simulink model "rns_sm"  (R2025b)
settings: Solver=ode45  StartTime=0.0  StopTime=T_END  MaxStep=0.01  RelTol=1e-10  AbsTol=1e-12
values from neighbouring files (symbols this model uses):
  a0 = 1    [run_rns_simscape.m]
  b0 = [a0/2 0]    [run_rns_simscape.m]
  I0 = m0*(a0^2 + a0^2)/12    (= 16.6666666667)    [run_rns_simscape.m]
  IN = MS.*LEN.^2/12    [run_rns_simscape.m]
  K_TH = 1.0    (= 1)    [run_rns_simscape.m]
  KP_EE = 2.0    (= 2)    [run_rns_simscape.m]
  LAM = 0.02    [run_rns_simscape.m]
  LEN = [1 1 0.5]    [run_rns_simscape.m]
  m = modelName    [build_rns_sm.m]
  m0 = 100    [run_rns_simscape.m]
  METHOD = cases{c, 2}    [run_rns_simscape.m]
  MS = [10 10 5]    [run_rns_simscape.m]
  QM0 = deg2rad([30 60 -45])    [run_rns_simscape.m]
  s = 10*x^3 - 15*x^4 + 6*x^5    [rns_controller.m]
  T_MOVE = 8    [run_rns_simscape.m]
  XG = goals.(cases{c, 1})    [run_rns_simscape.m]
  XS = d0(2:3).'    [run_rns_simscape.m]
  Y = squeeze(out.Y_sm)    [run_rns_simscape.m]
undefined symbols (not defined in the file or in its folder): X, Z
libraries: sm_lib x16, nesl_utility x10
settings Model: Creator=avaza  LastModifiedBy=avaza
settings DataIOCC: SaveOutput=off  TimeSaveName=t_sm  OutputOption=SpecifiedOutputTimes  OutputTimes=0:0.01:T_END
settings DebuggingCC: AlgebraicLoopMsg=none

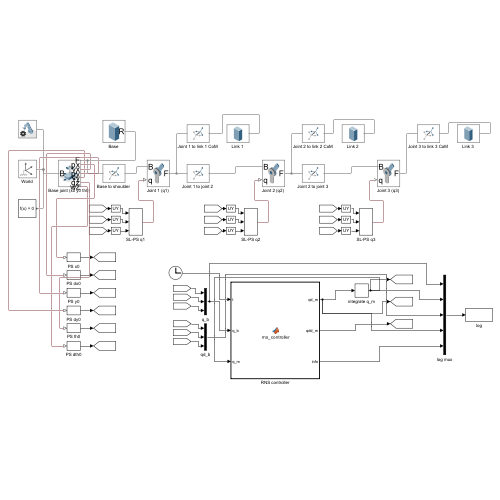
[thumbnail: Simulink's stored preview of the top-level diagram]
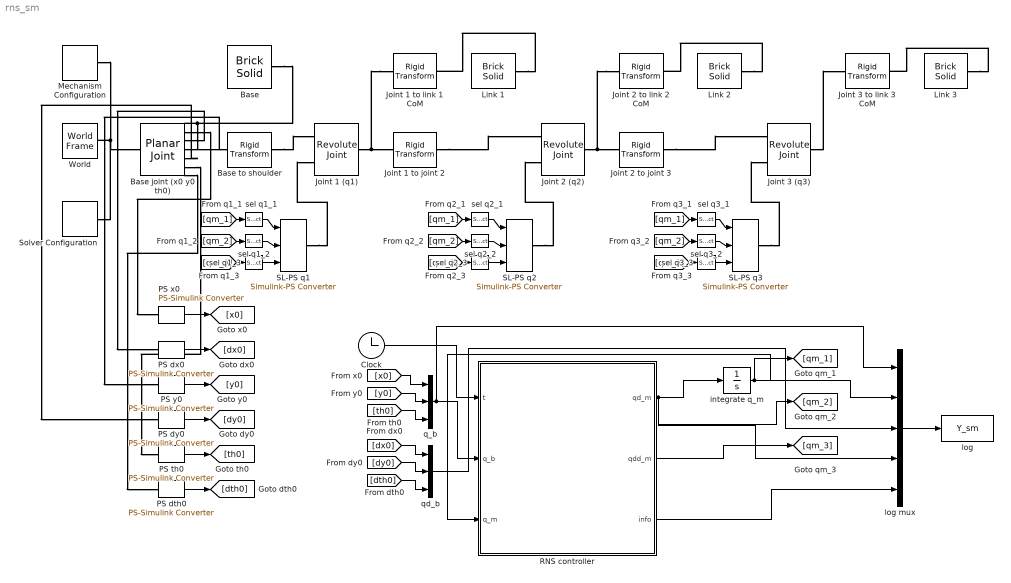
== system rns_sm ==
  Base : sm_lib/Body Elements/Brick Solid  BrickDimensions=[a0 a0 0.2]  BrickDimensionsUnits=m  ExportEntireGeometry=off  InertiaType=Custom  BasedOnType=Density  Density=1000  DensityUnits=kg/m^3  Mass=m0  MassUnits=kg  CenterOfMass=[0 0 0]  CenterOfMassUnits=m  MomentsOfInertia=[0.55*I0 0.55*I0 I0]  MomentsOfInertiaUnits=kg*m^2  ProductsOfInertia=[0 0 0]  ProductsOfInertiaUnits=kg*m^2  GraphicType=FromGeometry  MarkerShape=Sphere  MarkerSize=10  GraphicVisPropType=SimpleVisualProperties  GraphicDiffuseColor=[0.6 0.6 0.7]  GraphicOpacity=1  GraphicSpecularColor=[0.5 0.5 0.5 1.0]  GraphicAmbientColor=[0.15 0.15 0.15 1.0]  GraphicEmissiveColor=[0.0 0.0 0.0 1.0]  GraphicShininess=75  DoExposeReferenceFrame=on  SerializedFrames=<Frames/>
  Base joint (x0 y0 th0) : sm_lib/Joints/Planar Joint  JointMode=Normal  CompositeWrenchDir=FollowerOnBase  CompositeWrenchFrame=BaseFrame  SenseConstraintForce=off  SenseConstraintTorque=off  SenseTotalForce=off  SenseTotalTorque=off  PxPositionTargetSpecify=off  PxPositionTargetPriority=High  PxPositionTargetValue=0  PxPositionTargetValueUnits=m  PxVelocityTargetSpecify=off  PxVelocityTargetPriority=High  PxVelocityTargetValue=0  PxVelocityTargetValueUnits=m/s  PxEquilibriumPosition=0  PxEquilibriumPositionUnits=m  PxSpringStiffness=0  PxSpringStiffnessUnits=N/m  PxDampingCoefficient=0  PxDampingCoefficientUnits=N/(m/s)  PxLowerLimitSpecify=off  PxLowerLimitBound=-1  PxLowerLimitBoundUnits=m  PxLowerLimitStiffness=1e6  PxLowerLimitStiffnessUnits=N/m  PxLowerLimitDamping=1e3  PxLowerLimitDampingUnits=N/(m/s)  PxLowerLimitTransitionRegionWidth=1e-4  PxLowerLimitTransitionRegionWidthUnits=m  PxUpperLimitSpecify=off  PxUpperLimitBound=1  PxUpperLimitBoundUnits=m  PxUpperLimitStiffness=1e6  PxUpperLimitStiffnessUnits=N/m  PxUpperLimitDamping=1e3  PxUpperLimitDampingUnits=N/(m/s)  PxUpperLimitTransitionRegionWidth=1e-4  PxUpperLimitTransitionRegionWidthUnits=m  PxTorqueActuationMode=NoTorque  PxMotionActuationMode=ComputedMotion  PxSensePosition=on  PxSenseVelocity=on  PxSenseAcceleration=off  PxSenseTorqueForce=off  PxSenseLowerLimitTorqueForce=off  PxSenseUpperLimitTorqueForce=off  PyPositionTargetSpecify=off  PyPositionTargetPriority=High  PyPositionTargetValue=0  PyPositionTargetValueUnits=m  PyVelocityTargetSpecify=off  PyVelocityTargetPriority=High  PyVelocityTargetValue=0  PyVelocityTargetValueUnits=m/s  PyEquilibriumPosition=0  PyEquilibriumPositionUnits=m  PySpringStiffness=0  PySpringStiffnessUnits=N/m  PyDampingCoefficient=0  PyDampingCoefficientUnits=N/(m/s)  PyLowerLimitSpecify=off  PyLowerLimitBound=-1  PyLowerLimitBoundUnits=m  PyLowerLimitStiffness=1e6  PyLowerLimitStiffnessUnits=N/m  PyLowerLimitDamping=1e3  PyLowerLimitDampingUnits=N/(m/s)  PyLowerLimitTransitionRegionWidth=1e-4  PyLowerLimitTransitionRegionWidthUnits=m  PyUpperLimitSpecify=off  PyUpperLimitBound=1  PyUpperLimitBoundUnits=m  PyUpperLimitStiffness=1e6  PyUpperLimitStiffnessUnits=N/m  PyUpperLimitDamping=1e3  PyUpperLimitDampingUnits=N/(m/s)  PyUpperLimitTransitionRegionWidth=1e-4  PyUpperLimitTransitionRegionWidthUnits=m  PyTorqueActuationMode=NoTorque  PyMotionActuationMode=ComputedMotion  PySensePosition=on  PySenseVelocity=on  PySenseAcceleration=off  PySenseTorqueForce=off  PySenseLowerLimitTorqueForce=off  PySenseUpperLimitTorqueForce=off  RzPositionTargetSpecify=off  RzPositionTargetPriority=High  RzPositionTargetValue=0  RzPositionTargetValueUnits=deg  RzVelocityTargetSpecify=off  RzVelocityTargetPriority=High  RzVelocityTargetValue=0  RzVelocityTargetValueUnits=deg/s  RzEquilibriumPosition=0  RzEquilibriumPositionUnits=deg  RzSpringStiffness=0  RzSpringStiffnessUnits=N*m/deg  RzDampingCoefficient=0  RzDampingCoefficientUnits=N*m/(deg/s)  RzLowerLimitSpecify=off  RzLowerLimitBound=-90  RzLowerLimitBoundUnits=deg  RzLowerLimitStiffness=1e4  RzLowerLimitStiffnessUnits=N*m/deg  RzLowerLimitDamping=10  RzLowerLimitDampingUnits=N*m/(deg/s)  RzLowerLimitTransitionRegionWidth=0.1  RzLowerLimitTransitionRegionWidthUnits=deg  RzUpperLimitSpecify=off  RzUpperLimitBound=90  RzUpperLimitBoundUnits=deg  RzUpperLimitStiffness=1e4  RzUpperLimitStiffnessUnits=N*m/deg  RzUpperLimitDamping=10  RzUpperLimitDampingUnits=N*m/(deg/s)  RzUpperLimitTransitionRegionWidth=0.1  RzUpperLimitTransitionRegionWidthUnits=deg  RzTorqueActuationMode=NoTorque  RzMotionActuationMode=ComputedMotion  RzSensePosition=on  RzSenseVelocity=on  RzSenseAcceleration=off  RzSenseTorqueForce=off  RzSenseLowerLimitTorqueForce=off  RzSenseUpperLimitTorqueForce=off
  Base to shoulder : sm_lib/Frames and Transforms/Rigid Transform  RotationMethod=None  FollAlignAxisA=+X  BaseAlignAxisA=+Y  FollAlignAxisB=+Y  BaseAlignAxisB=+Z  RotationStandardAxis=+Z  RotationAngle=0  RotationAngleUnits=deg  RotationArbitraryAxis=[0 0 1]  RotationSequenceAxes=FollowerAxes  RotationSequence=XYX  RotationSequenceAngles=[0 0 0]  RotationSequenceAnglesUnits=deg  RotationMatrix=[1 0 0;0 1 0;0 0 1]  Quaternion=[1 0 0 0]  TranslationMethod=Cartesian  TranslationCartesianOffset=[b0(1) b0(2) 0]  TranslationCartesianOffsetUnits=m  TranslationStandardAxis=+Z  TranslationStandardOffset=0  TranslationStandardOffsetUnits=m  TranslationROffset=0  TranslationROffsetUnits=m  TranslationThetaOffset=0  TranslationThetaOffsetUnits=deg  TranslationZOffset=0  TranslationZOffsetUnits=m
  Clock : Clock
  Joint 1 (q1) : sm_lib/Joints/Revolute Joint  JointMode=Normal  CompositeWrenchDir=FollowerOnBase  CompositeWrenchFrame=BaseFrame  SenseConstraintForce=off  SenseConstraintTorque=off  SenseTotalForce=off  SenseTotalTorque=off  PositionTargetSpecify=off  PositionTargetPriority=High  PositionTargetValue=0  PositionTargetValueUnits=deg  VelocityTargetSpecify=off  VelocityTargetPriority=High  VelocityTargetValue=0  VelocityTargetValueUnits=deg/s  EquilibriumPosition=0  EquilibriumPositionUnits=deg  SpringStiffness=0  SpringStiffnessUnits=N*m/deg  DampingCoefficient=0  DampingCoefficientUnits=N*m/(deg/s)  LowerLimitSpecify=off  LowerLimitBound=-90  LowerLimitBoundUnits=deg  LowerLimitStiffness=1e4  LowerLimitStiffnessUnits=N*m/deg  LowerLimitDamping=10  LowerLimitDampingUnits=N*m/(deg/s)  LowerLimitTransitionRegionWidth=0.1  LowerLimitTransitionRegionWidthUnits=deg  UpperLimitSpecify=off  UpperLimitBound=90  UpperLimitBoundUnits=deg  UpperLimitStiffness=1e4  UpperLimitStiffnessUnits=N*m/deg  UpperLimitDamping=10  UpperLimitDampingUnits=N*m/(deg/s)  UpperLimitTransitionRegionWidth=0.1  UpperLimitTransitionRegionWidthUnits=deg  TorqueActuationMode=ComputedTorque  MotionActuationMode=InputMotion  SensePosition=off  SenseVelocity=off  SenseAcceleration=off  SenseTorqueForce=off  SenseLowerLimitTorqueForce=off  SenseUpperLimitTorqueForce=off
  Joint 1 to joint 2 : sm_lib/Frames and Transforms/Rigid Transform  RotationMethod=None  FollAlignAxisA=+X  BaseAlignAxisA=+Y  FollAlignAxisB=+Y  BaseAlignAxisB=+Z  RotationStandardAxis=+Z  RotationAngle=0  RotationAngleUnits=deg  RotationArbitraryAxis=[0 0 1]  RotationSequenceAxes=FollowerAxes  RotationSequence=XYX  RotationSequenceAngles=[0 0 0]  RotationSequenceAnglesUnits=deg  RotationMatrix=[1 0 0;0 1 0;0 0 1]  Quaternion=[1 0 0 0]  TranslationMethod=Cartesian  TranslationCartesianOffset=[LEN(1) 0 0]  TranslationCartesianOffsetUnits=m  TranslationStandardAxis=+Z  TranslationStandardOffset=0  TranslationStandardOffsetUnits=m  TranslationROffset=0  TranslationROffsetUnits=m  TranslationThetaOffset=0  TranslationThetaOffsetUnits=deg  TranslationZOffset=0  TranslationZOffsetUnits=m
  Joint 1 to link 1 CoM : sm_lib/Frames and Transforms/Rigid Transform  RotationMethod=None  FollAlignAxisA=+X  BaseAlignAxisA=+Y  FollAlignAxisB=+Y  BaseAlignAxisB=+Z  RotationStandardAxis=+Z  RotationAngle=0  RotationAngleUnits=deg  RotationArbitraryAxis=[0 0 1]  RotationSequenceAxes=FollowerAxes  RotationSequence=XYX  RotationSequenceAngles=[0 0 0]  RotationSequenceAnglesUnits=deg  RotationMatrix=[1 0 0;0 1 0;0 0 1]  Quaternion=[1 0 0 0]  TranslationMethod=Cartesian  TranslationCartesianOffset=[LEN(1)/2 0 0]  TranslationCartesianOffsetUnits=m  TranslationStandardAxis=+Z  TranslationStandardOffset=0  TranslationStandardOffsetUnits=m  TranslationROffset=0  TranslationROffsetUnits=m  TranslationThetaOffset=0  TranslationThetaOffsetUnits=deg  TranslationZOffset=0  TranslationZOffsetUnits=m
  Joint 2 (q2) : sm_lib/Joints/Revolute Joint  JointMode=Normal  CompositeWrenchDir=FollowerOnBase  CompositeWrenchFrame=BaseFrame  SenseConstraintForce=off  SenseConstraintTorque=off  SenseTotalForce=off  SenseTotalTorque=off  PositionTargetSpecify=off  PositionTargetPriority=High  PositionTargetValue=0  PositionTargetValueUnits=deg  VelocityTargetSpecify=off  VelocityTargetPriority=High  VelocityTargetValue=0  VelocityTargetValueUnits=deg/s  EquilibriumPosition=0  EquilibriumPositionUnits=deg  SpringStiffness=0  SpringStiffnessUnits=N*m/deg  DampingCoefficient=0  DampingCoefficientUnits=N*m/(deg/s)  LowerLimitSpecify=off  LowerLimitBound=-90  LowerLimitBoundUnits=deg  LowerLimitStiffness=1e4  LowerLimitStiffnessUnits=N*m/deg  LowerLimitDamping=10  LowerLimitDampingUnits=N*m/(deg/s)  LowerLimitTransitionRegionWidth=0.1  LowerLimitTransitionRegionWidthUnits=deg  UpperLimitSpecify=off  UpperLimitBound=90  UpperLimitBoundUnits=deg  UpperLimitStiffness=1e4  UpperLimitStiffnessUnits=N*m/deg  UpperLimitDamping=10  UpperLimitDampingUnits=N*m/(deg/s)  UpperLimitTransitionRegionWidth=0.1  UpperLimitTransitionRegionWidthUnits=deg  TorqueActuationMode=ComputedTorque  MotionActuationMode=InputMotion  SensePosition=off  SenseVelocity=off  SenseAcceleration=off  SenseTorqueForce=off  SenseLowerLimitTorqueForce=off  SenseUpperLimitTorqueForce=off
  Joint 2 to joint 3 : sm_lib/Frames and Transforms/Rigid Transform  RotationMethod=None  FollAlignAxisA=+X  BaseAlignAxisA=+Y  FollAlignAxisB=+Y  BaseAlignAxisB=+Z  RotationStandardAxis=+Z  RotationAngle=0  RotationAngleUnits=deg  RotationArbitraryAxis=[0 0 1]  RotationSequenceAxes=FollowerAxes  RotationSequence=XYX  RotationSequenceAngles=[0 0 0]  RotationSequenceAnglesUnits=deg  RotationMatrix=[1 0 0;0 1 0;0 0 1]  Quaternion=[1 0 0 0]  TranslationMethod=Cartesian  TranslationCartesianOffset=[LEN(2) 0 0]  TranslationCartesianOffsetUnits=m  TranslationStandardAxis=+Z  TranslationStandardOffset=0  TranslationStandardOffsetUnits=m  TranslationROffset=0  TranslationROffsetUnits=m  TranslationThetaOffset=0  TranslationThetaOffsetUnits=deg  TranslationZOffset=0  TranslationZOffsetUnits=m
  Joint 2 to link 2 CoM : sm_lib/Frames and Transforms/Rigid Transform  RotationMethod=None  FollAlignAxisA=+X  BaseAlignAxisA=+Y  FollAlignAxisB=+Y  BaseAlignAxisB=+Z  RotationStandardAxis=+Z  RotationAngle=0  RotationAngleUnits=deg  RotationArbitraryAxis=[0 0 1]  RotationSequenceAxes=FollowerAxes  RotationSequence=XYX  RotationSequenceAngles=[0 0 0]  RotationSequenceAnglesUnits=deg  RotationMatrix=[1 0 0;0 1 0;0 0 1]  Quaternion=[1 0 0 0]  TranslationMethod=Cartesian  TranslationCartesianOffset=[LEN(2)/2 0 0]  TranslationCartesianOffsetUnits=m  TranslationStandardAxis=+Z  TranslationStandardOffset=0  TranslationStandardOffsetUnits=m  TranslationROffset=0  TranslationROffsetUnits=m  TranslationThetaOffset=0  TranslationThetaOffsetUnits=deg  TranslationZOffset=0  TranslationZOffsetUnits=m
  Joint 3 (q3) : sm_lib/Joints/Revolute Joint  JointMode=Normal  CompositeWrenchDir=FollowerOnBase  CompositeWrenchFrame=BaseFrame  SenseConstraintForce=off  SenseConstraintTorque=off  SenseTotalForce=off  SenseTotalTorque=off  PositionTargetSpecify=off  PositionTargetPriority=High  PositionTargetValue=0  PositionTargetValueUnits=deg  VelocityTargetSpecify=off  VelocityTargetPriority=High  VelocityTargetValue=0  VelocityTargetValueUnits=deg/s  EquilibriumPosition=0  EquilibriumPositionUnits=deg  SpringStiffness=0  SpringStiffnessUnits=N*m/deg  DampingCoefficient=0  DampingCoefficientUnits=N*m/(deg/s)  LowerLimitSpecify=off  LowerLimitBound=-90  LowerLimitBoundUnits=deg  LowerLimitStiffness=1e4  LowerLimitStiffnessUnits=N*m/deg  LowerLimitDamping=10  LowerLimitDampingUnits=N*m/(deg/s)  LowerLimitTransitionRegionWidth=0.1  LowerLimitTransitionRegionWidthUnits=deg  UpperLimitSpecify=off  UpperLimitBound=90  UpperLimitBoundUnits=deg  UpperLimitStiffness=1e4  UpperLimitStiffnessUnits=N*m/deg  UpperLimitDamping=10  UpperLimitDampingUnits=N*m/(deg/s)  UpperLimitTransitionRegionWidth=0.1  UpperLimitTransitionRegionWidthUnits=deg  TorqueActuationMode=ComputedTorque  MotionActuationMode=InputMotion  SensePosition=off  SenseVelocity=off  SenseAcceleration=off  SenseTorqueForce=off  SenseLowerLimitTorqueForce=off  SenseUpperLimitTorqueForce=off
  Joint 3 to link 3 CoM : sm_lib/Frames and Transforms/Rigid Transform  RotationMethod=None  FollAlignAxisA=+X  BaseAlignAxisA=+Y  FollAlignAxisB=+Y  BaseAlignAxisB=+Z  RotationStandardAxis=+Z  RotationAngle=0  RotationAngleUnits=deg  RotationArbitraryAxis=[0 0 1]  RotationSequenceAxes=FollowerAxes  RotationSequence=XYX  RotationSequenceAngles=[0 0 0]  RotationSequenceAnglesUnits=deg  RotationMatrix=[1 0 0;0 1 0;0 0 1]  Quaternion=[1 0 0 0]  TranslationMethod=Cartesian  TranslationCartesianOffset=[LEN(3)/2 0 0]  TranslationCartesianOffsetUnits=m  TranslationStandardAxis=+Z  TranslationStandardOffset=0  TranslationStandardOffsetUnits=m  TranslationROffset=0  TranslationROffsetUnits=m  TranslationThetaOffset=0  TranslationThetaOffsetUnits=deg  TranslationZOffset=0  TranslationZOffsetUnits=m
  Link 1 : sm_lib/Body Elements/Brick Solid  BrickDimensions=[LEN(1) 0.08 0.08]  BrickDimensionsUnits=m  ExportEntireGeometry=off  InertiaType=Custom  BasedOnType=Density  Density=1000  DensityUnits=kg/m^3  Mass=MS(1)  MassUnits=kg  CenterOfMass=[0 0 0]  CenterOfMassUnits=m  MomentsOfInertia=[0.01 IN(1) IN(1)]  MomentsOfInertiaUnits=kg*m^2  ProductsOfInertia=[0 0 0]  ProductsOfInertiaUnits=kg*m^2  GraphicType=FromGeometry  MarkerShape=Sphere  MarkerSize=10  GraphicVisPropType=SimpleVisualProperties  GraphicDiffuseColor=[0.85 0.45 0.2]  GraphicOpacity=1  GraphicSpecularColor=[0.5 0.5 0.5 1.0]  GraphicAmbientColor=[0.15 0.15 0.15 1.0]  GraphicEmissiveColor=[0.0 0.0 0.0 1.0]  GraphicShininess=75  DoExposeReferenceFrame=on  SerializedFrames=<Frames/>
  Link 2 : sm_lib/Body Elements/Brick Solid  BrickDimensions=[LEN(2) 0.08 0.08]  BrickDimensionsUnits=m  ExportEntireGeometry=off  InertiaType=Custom  BasedOnType=Density  Density=1000  DensityUnits=kg/m^3  Mass=MS(2)  MassUnits=kg  CenterOfMass=[0 0 0]  CenterOfMassUnits=m  MomentsOfInertia=[0.01 IN(2) IN(2)]  MomentsOfInertiaUnits=kg*m^2  ProductsOfInertia=[0 0 0]  ProductsOfInertiaUnits=kg*m^2  GraphicType=FromGeometry  MarkerShape=Sphere  MarkerSize=10  GraphicVisPropType=SimpleVisualProperties  GraphicDiffuseColor=[0.2 0.5 0.85]  GraphicOpacity=1  GraphicSpecularColor=[0.5 0.5 0.5 1.0]  GraphicAmbientColor=[0.15 0.15 0.15 1.0]  GraphicEmissiveColor=[0.0 0.0 0.0 1.0]  GraphicShininess=75  DoExposeReferenceFrame=on  SerializedFrames=<Frames/>
  Link 3 : sm_lib/Body Elements/Brick Solid  BrickDimensions=[LEN(3) 0.08 0.08]  BrickDimensionsUnits=m  ExportEntireGeometry=off  InertiaType=Custom  BasedOnType=Density  Density=1000  DensityUnits=kg/m^3  Mass=MS(3)  MassUnits=kg  CenterOfMass=[0 0 0]  CenterOfMassUnits=m  MomentsOfInertia=[0.01 IN(3) IN(3)]  MomentsOfInertiaUnits=kg*m^2  ProductsOfInertia=[0 0 0]  ProductsOfInertiaUnits=kg*m^2  GraphicType=FromGeometry  MarkerShape=Sphere  MarkerSize=10  GraphicVisPropType=SimpleVisualProperties  GraphicDiffuseColor=[0.3 0.7 0.3]  GraphicOpacity=1  GraphicSpecularColor=[0.5 0.5 0.5 1.0]  GraphicAmbientColor=[0.15 0.15 0.15 1.0]  GraphicEmissiveColor=[0.0 0.0 0.0 1.0]  GraphicShininess=75  DoExposeReferenceFrame=on  SerializedFrames=<Frames/>
  Mechanism Configuration : sm_lib/Utilities/Mechanism Configuration  UniformGravity=None  GravityVector=[0 0 -9.80665]  GravityVectorUnits=m/s^2  LinearizationDelta=0.001  JointModeTransitionNonlinearIterations=2
  PS dth0 : nesl_utility/PS-Simulink Converter  PhysicalDomain=network_engine_domain  SubClassName=ps_output  LeftPortType=input  RightPortType=output  PseudoPeriodic=off  Frequencies=[]  VectorFormat=inherit  Unit=rad/s  AffineConversion=off
  PS dx0 : nesl_utility/PS-Simulink Converter  PhysicalDomain=network_engine_domain  SubClassName=ps_output  LeftPortType=input  RightPortType=output  PseudoPeriodic=off  Frequencies=[]  VectorFormat=inherit  Unit=m/s  AffineConversion=off
  PS dy0 : nesl_utility/PS-Simulink Converter  PhysicalDomain=network_engine_domain  SubClassName=ps_output  LeftPortType=input  RightPortType=output  PseudoPeriodic=off  Frequencies=[]  VectorFormat=inherit  Unit=m/s  AffineConversion=off
  PS th0 : nesl_utility/PS-Simulink Converter  PhysicalDomain=network_engine_domain  SubClassName=ps_output  LeftPortType=input  RightPortType=output  PseudoPeriodic=off  Frequencies=[]  VectorFormat=inherit  Unit=rad  AffineConversion=off
  PS x0 : nesl_utility/PS-Simulink Converter  PhysicalDomain=network_engine_domain  SubClassName=ps_output  LeftPortType=input  RightPortType=output  PseudoPeriodic=off  Frequencies=[]  VectorFormat=inherit  Unit=m  AffineConversion=off
  PS y0 : nesl_utility/PS-Simulink Converter  PhysicalDomain=network_engine_domain  SubClassName=ps_output  LeftPortType=input  RightPortType=output  PseudoPeriodic=off  Frequencies=[]  VectorFormat=inherit  Unit=m  AffineConversion=off
  RNS controller : MATLAB Function  TreatAsAtomicUnit=on
  SL-PS q1 : nesl_utility/Simulink-PS Converter  PhysicalDomain=network_engine_domain  SubClassName=ps_input  LeftPortType=input  RightPortType=output  PseudoPeriodic=off  Frequencies=[]  NoiseDistribution=none  NoiseParameters=[]  Unit=rad  AffineConversion=off  FilteringAndDerivatives=provide  SimscapeFilterOrder=1  InputFilterTimeConstant=0.001  UdotUserProvided=2
  SL-PS q2 : nesl_utility/Simulink-PS Converter  PhysicalDomain=network_engine_domain  SubClassName=ps_input  LeftPortType=input  RightPortType=output  PseudoPeriodic=off  Frequencies=[]  NoiseDistribution=none  NoiseParameters=[]  Unit=rad  AffineConversion=off  FilteringAndDerivatives=provide  SimscapeFilterOrder=1  InputFilterTimeConstant=0.001  UdotUserProvided=2
  SL-PS q3 : nesl_utility/Simulink-PS Converter  PhysicalDomain=network_engine_domain  SubClassName=ps_input  LeftPortType=input  RightPortType=output  PseudoPeriodic=off  Frequencies=[]  NoiseDistribution=none  NoiseParameters=[]  Unit=rad  AffineConversion=off  FilteringAndDerivatives=provide  SimscapeFilterOrder=1  InputFilterTimeConstant=0.001  UdotUserProvided=2
  Solver Configuration : nesl_utility/Solver Configuration  PhysicalDomain=network_engine_domain  SubClassName=solver  LeftPortType=input  RightPortType=generic  Tones=[]  Harmonics=[]  SimulateNoise=off  Profile=off  UseLocalSampling=off  EnableSwitchedLinearOptims=on  FrequencyDomain=off  UseCCode=off  RelTol=0.001  AbsTol=0.001  MinStep=1e-09  ToWorkspace=off  RevertToSquareIcSolve=off  NumHomotopyIterations=100  PhasorMode=off  PhasorModeNumHarmonics=1  ConsistencySolver=NEWTON_XTOL_AFTER_FTOL  IndexReductionMethod=DerivativeReplacement  DoDC=off  ResidualTolerance=1e-09  ConsistencyTolSource=GLOBAL  ConsistencyAbsTol=0.001  ConsistencyRelTol=0.001  ConsistencyTolFactor=0.001  UseLocalSolver=off  LocalSolverChoice=NE_BACKWARD_EULER_ADVANCER  ResolveIndetEquations=on  FunctionEvalNumThread=1  LocalSolverSampleTime=0.001  DoFixedCost=off  MaxNonlinIter=3  MaxModeIter=2  ComputeImpulses=off  ImpulseIterations=2  LinearAlgebra=auto  LinearAlgebraNumThread=0  EquationFormulation=NE_TIME_EF  DelaysMemoryBudget=1024  AutomaticFiltering=on  FilteringTimeConstant=0.001  PartitionStorageMethod=AS_NEEDED  PartitionMemoryBudget=1024  PartitionMethod=ROBUST  MultibodyUseLocalSolver=off  MultibodyLocalSolverChoice=ODE1  MultibodyLocalSolverSampleTime=0.001
  World : sm_lib/Frames and Transforms/World Frame
  integrate q_m : Integrator  InitialCondition=QM0(:)
  log : ToWorkspace  VariableName=Y_sm  SampleTime=-1
  log mux : Mux  Inputs=5
  q_b : Mux  Inputs=3
  qd_b : Mux  Inputs=3
  sel q1_1 : Selector  InputPortWidth=3  IndexOptions=Index vector (dialog)  Indices=1  OutputSizes=1
  sel q1_2 : Selector  InputPortWidth=3  IndexOptions=Index vector (dialog)  Indices=1  OutputSizes=1
  sel q1_3 : Selector  InputPortWidth=3  IndexOptions=Index vector (dialog)  Indices=1  OutputSizes=1
  sel q2_1 : Selector  InputPortWidth=3  IndexOptions=Index vector (dialog)  Indices=2  OutputSizes=1
  sel q2_2 : Selector  InputPortWidth=3  IndexOptions=Index vector (dialog)  Indices=2  OutputSizes=1
  sel q2_3 : Selector  InputPortWidth=3  IndexOptions=Index vector (dialog)  Indices=2  OutputSizes=1
  sel q3_1 : Selector  InputPortWidth=3  IndexOptions=Index vector (dialog)  Indices=3  OutputSizes=1
  sel q3_2 : Selector  InputPortWidth=3  IndexOptions=Index vector (dialog)  Indices=3  OutputSizes=1
  sel q3_3 : Selector  InputPortWidth=3  IndexOptions=Index vector (dialog)  Indices=3  OutputSizes=1
  wires:
  [qm_1] -> sel q1_1/1
  sel q1_1/1 -> SL-PS q1/1
  [qm_2] -> sel q1_2/1
  sel q1_2/1 -> SL-PS q1/2
  [qm_3] -> sel q1_3/1
  sel q1_3/1 -> SL-PS q1/3
  [qm_1] -> sel q2_1/1
  sel q2_1/1 -> SL-PS q2/1
  [qm_2] -> sel q2_2/1
  sel q2_2/1 -> SL-PS q2/2
  [qm_3] -> sel q2_3/1
  sel q2_3/1 -> SL-PS q2/3
  [qm_1] -> sel q3_1/1
  sel q3_1/1 -> SL-PS q3/1
  [qm_2] -> sel q3_2/1
  sel q3_2/1 -> SL-PS q3/2
  [qm_3] -> sel q3_3/1
  sel q3_3/1 -> SL-PS q3/3
  PS x0/1 -> [x0]
  PS dx0/1 -> [dx0]
  PS y0/1 -> [y0]
  PS dy0/1 -> [dy0]
  PS th0/1 -> [th0]
  PS dth0/1 -> [dth0]
  [x0] -> q_b/1
  [dx0] -> qd_b/1
  [y0] -> q_b/2
  [dy0] -> qd_b/2
  [th0] -> q_b/3
  [dth0] -> qd_b/3
  Clock/1 -> RNS controller/1(t)
  q_b/1 -> RNS controller/2(q_b), log mux/1
  integrate q_m/1 -> RNS controller/3(q_m), [qm_1], log mux/2
  RNS controller/1(qd_m) -> integrate q_m/1, [qm_2], log mux/4
  RNS controller/2(qdd_m) -> [qm_3]
  qd_b/1 -> log mux/3
  RNS controller/3(info) -> log mux/5
  log mux/1 -> log/1
  connections:
  Mechanism Configuration/RConn1 -- Solver Configuration/RConn1 -- World/RConn1 -- Base joint (x0 y0 th0)/LConn1
  Base joint (x0 y0 th0)/RConn1 -- Base/RConn1 -- Base to shoulder/LConn1
  Base to shoulder/RConn1 -- Joint 1 (q1)/LConn1
  Joint 1 to link 1 CoM/LConn1 -- Joint 1 (q1)/RConn1 -- Joint 1 to joint 2/LConn1
  Link 1/RConn1 -- Joint 1 to link 1 CoM/RConn1
  SL-PS q1/RConn1 -- Joint 1 (q1)/LConn2
  Joint 1 to joint 2/RConn1 -- Joint 2 (q2)/LConn1
  Joint 2 to link 2 CoM/LConn1 -- Joint 2 (q2)/RConn1 -- Joint 2 to joint 3/LConn1
  Link 2/RConn1 -- Joint 2 to link 2 CoM/RConn1
  SL-PS q2/RConn1 -- Joint 2 (q2)/LConn2
  Joint 2 to joint 3/RConn1 -- Joint 3 (q3)/LConn1
  Joint 3 (q3)/RConn1 -- Joint 3 to link 3 CoM/LConn1
  Link 3/RConn1 -- Joint 3 to link 3 CoM/RConn1
  SL-PS q3/RConn1 -- Joint 3 (q3)/LConn2
  Base joint (x0 y0 th0)/RConn2 -- PS x0/LConn1
  Base joint (x0 y0 th0)/RConn3 -- PS dx0/LConn1
  Base joint (x0 y0 th0)/RConn4 -- PS y0/LConn1
  Base joint (x0 y0 th0)/RConn5 -- PS dy0/LConn1
  Base joint (x0 y0 th0)/RConn6 -- PS th0/LConn1
  Base joint (x0 y0 th0)/RConn7 -- PS dth0/LConn1

== matlab function rns_sm/RNS controller ==
  data: t input; qd_m output; q_b input; q_m input; qdd_m output; info output; LEN parameter; MS parameter; IN parameter; m0 parameter; I0 parameter; b0 parameter; KP_EE parameter; K_TH parameter; LAM parameter; METHOD parameter; XS parameter; XG parameter; T_MOVE parameter
function [qd_m, qdd_m, info] = rns_controller(t, q_b, q_m, LEN, MS, IN, m0, I0, b0, ...
KP_EE, K_TH, LAM, METHOD, XS, XG, T_MOVE)
%RNS_CONTROLLER  Joint-rate command of project 1b (same law as path_tracking.py).
%
%   Inputs: time, MEASURED base pose q_b = [x0 y0 th0] (from Simscape), joint angles q_m. Outputs: joint rates qd_m, their time derivative qdd_m (needed to
%   drive the Simscape joints by motion) and info = [det A; end-effector x; y].
%
%   METHOD: 0 = min-norm (base ignored), 1 = exact RNS, 2 = task priority + damped RNS.
%   The inertia matrix is computed numerically from the body Jacobians here; it is the
%   controller's MODEL. The plant (how the base really reacts) is Simscape's.

q = [q_b(:); q_m(:)];
[qd_m, detA, xe, B] = law(q, t, LEN, MS, IN, m0, I0, b0, KP_EE, K_TH, LAM, METHOD, XS, XG, T_MOVE);
% time derivative of the law along the motion (central difference). The base rates here
% are the controller's own zero-momentum prediction B*qd_m, so the feedforward does not
% depend on the plant's instantaneous velocity response.
qd = [B*qd_m; qd_m];
h = 1e-5;
qp = law(q + h*qd, t + h, LEN, MS, IN, m0, I0, b0, KP_EE, K_TH, LAM, METHOD, XS, XG, T_MOVE);
qn = law(q - h*qd, t - h, LEN, MS, IN, m0, I0, b0, KP_EE, K_TH, LAM, METHOD, XS, XG, T_MOVE);
qdd_m = (qp - qn) / (2*h);
info = [detA; xe];
end

function [qd_m, detA, xe, B] = law(q, t, LEN, MS, IN, m0, I0, b0, KP_EE, K_TH, LAM, METHOD, XS, XG, T_MOVE)
[M, xe, Je] = kin(q, LEN, MS, IN, m0, I0, b0);
B = -M(1:3, 1:3) \ M(1:3, 4:6);            % base rates per unit joint rate (zero momentum)
b = B(3, :);                               % reaction row: w0 = b qd_m
Js = Je(:, 4:6) + Je(:, 1:3) * B;          % generalized Jacobian J*
% straight-line quintic reference
x = min(max(t / T_MOVE, 0), 1);
s = 10*x^3 - 15*x^4 + 6*x^5;
ds = 0;
if t >= 0 && t < T_MOVE, ds = (30*x^2 - 60*x^3 + 30*x^4) / T_MOVE; end
xd = XS(:) + s*(XG(:) - XS(:));
vd = ds*(XG(:) - XS(:));
v = vd + KP_EE*(xd - xe);
n = cross(Js(1, :).', Js(2, :).');          % null space of J*
detA = b * n;
qd0 = pinv(Js) * v;
w_c = -K_TH * q(3);
if METHOD == 0
    sn = 0;
elseif METHOD == 1
    sn = (w_c - b*qd0) / detA;
else
    sn = detA * (w_c - b*qd0) / (detA^2 + LAM^2);
end
qd_m = qd0 + sn*n;
end

function [M, xe, Je] = kin(q, LEN, MS, IN, m0, I0, b0)
% Mass matrix from the body Jacobians, M = sum(m Jv'Jv + I Jw'Jw), and the
% end-effector position + Jacobian. q = [x0 y0 th0 q1 q2 q3].
th = q(3);
phi = th + cumsum(q(4:6));
R = [cos(th) -sin(th); sin(th) cos(th)];
j1 = q(1:2) + R*b0(:);
dj1 = R*[-b0(2); b0(1)];                   % d(shoulder)/d th0
Jv0 = [eye(2), zeros(2, 4)];
Jw0 = [0 0 1 0 0 0];
M = m0*(Jv0.'*Jv0) + I0*(Jw0.'*Jw0);
xe = zeros(2, 1);
Je = zeros(2, 6);
for i = 1:4                                % i = 1..3 link CoMs, i = 4 end effector
    Jv = [eye(2), dj1, zeros(2, 3)];
    p = j1;
    last = min(i, 3);
    for k = 1:last
        lever = LEN(k);
        if i <= 3 && k == i, lever = LEN(k)/2; end
        nk = [-sin(phi(k)); cos(phi(k))];
        p = p + lever*[cos(phi(k)); sin(phi(k))];
        Jv(:, 3) = Jv(:, 3) + lever*nk;
        Jv(:, 4:3+k) = Jv(:, 4:3+k) + lever*nk*ones(1, k);
    end
    if i <= 3
        Jw = [0 0 1, ones(1, i), zeros(1, 3-i)];
        M = M + MS(i)*(Jv.'*Jv) + IN(i)*(Jw.'*Jw);
    else
        xe = p;
        Je = Jv;
    end
end
end
